simulink model "Quadruped_view"  (R2026a)
settings: Solver=ode23tb  StopTime=50
values from neighbouring files (symbols this model uses):
  a_amp = 0.03    [initializeRobotParameters.m]
  b_amp = 0.03    [initializeRobotParameters.m]
  dTheta = 20*pi/180    (= 0.349065850399)    [initializeRobotParameters.m]
  friction_force_max = mu_static * normal_force_max    [initializeRobotParameters.m]
  g = -9.81    [initializeRobotParameters.m]
  h_final = 0.2    [initializeRobotParameters.m]
  hip_eq_angle = 0    [initializeRobotParameters.m]
  init_ang_FL = d2r * quadrupedInverseKinematics(init_foot_disp_x,-init_body_height,l1,l2)    [initializeRobotParameters.m]
  init_ang_FR = init_ang_FL    [initializeRobotParameters.m]
  init_ang_RL = init_ang_FL    [initializeRobotParameters.m]
  init_ang_RR = init_ang_FL    [initializeRobotParameters.m]
  knee_eq_angle = 0    [initializeRobotParameters.m]
  l1 = 0.1422    [initializeRobotParameters.m]
  l2 = 0.115    [initializeRobotParameters.m]
  L_back = 0.305    [initializeRobotParameters.m]
  M = 1.318    [initializeRobotParameters.m]
  m1 = 0.17824    [initializeRobotParameters.m]
  m2 = 0.03558    [initializeRobotParameters.m]
  normal_force_max = ((M+4*m1+4*m2)*abs(g))/4    [initializeRobotParameters.m]
  period = 0.8    [initializeRobotParameters.m]
  pitch_max = 10 * d2r    (= 0.174532925199)    [initializeRobotParameters.m]
  q_hip_max = -30 * d2r    (= -0.523598775598)    [initializeRobotParameters.m]
  q_hip_min = -120 * d2r    (= -2.09439510239)    [initializeRobotParameters.m]
  q_knee_max = 140 * d2r    (= 2.44346095279)    [initializeRobotParameters.m]
  q_knee_min = 60 * d2r    (= 1.0471975512)    [initializeRobotParameters.m]
  roll_max = 10 * d2r    (= 0.174532925199)    [initializeRobotParameters.m]
  Tf = 10    [initializeRobotParameters.m]
  torso_dim = [L_back 0.04875 0.152]    [initializeRobotParameters.m]
  Tp = 0.15    [initializeRobotParameters.m]
  Ts = 0.025    [initializeRobotParameters.m]
  vx_max = 2.5    [initializeRobotParameters.m]
  vy_max = 2.5    [initializeRobotParameters.m]
  vz_max = 2.5    [initializeRobotParameters.m]
  w_max = 2*pi*60/60    (= 6.28318530718)    [initializeRobotParameters.m]
  y_init = init_body_height + foot_height    [initializeRobotParameters.m]
  y_max = l1*cos(q_hip_max) + l2*cos(q_hip_max+q_knee_min)    [initializeRobotParameters.m]
  y_min = 0.5    [initializeRobotParameters.m]
  yaw_max = 20 * d2r    (= 0.349065850399)    [initializeRobotParameters.m]
  z_max = 0.5    [initializeRobotParameters.m]
undefined symbols (not defined in the file or in its folder): Extr_Data_LinkEndHole, Extr_Data_Mesh, ground, joint, X, Y, Z
libraries: sm_lib x118, nesl_utility x54, simulink x4
(part 5 of 5)

== system Quadruped_view/Quadruped Robot/Leg RR/Lower Leg ==
  note: Geometry Only
  Cap F : sm_lib/Body Elements/Extruded Solid  ExtrusionType=General  PolygonNumSides=3  PolygonOuterRadius=1  PolygonOuterRadiusUnits=m  ExportEntireGeometry=off  ExtrusionCrossSection=Extr_Data_LinkEndHole(l2*0.1,l1*0.025,0.05*l2)  ExtrusionCrossSectionUnits=m  ExportConvexHullGeometry=off  ExtrusionLength=l2*0.1/3  ExtrusionLengthUnits=m  InertiaType=CalculateFromGeometry  BasedOnType=Density  Density=0  DensityUnits=kg/m^3  Mass=1  MassUnits=kg  CenterOfMass=[0 0 0]  CenterOfMassUnits=m  MomentsOfInertia=[1 1 1]  MomentsOfInertiaUnits=kg*m^2  ProductsOfInertia=[1 1 1]  ProductsOfInertiaUnits=kg*m^2  GraphicType=FromGeometry  MarkerShape=Sphere  MarkerSize=10  GraphicVisPropType=SimpleVisualProperties  GraphicDiffuseColor=[164 184 200]/255  GraphicOpacity=1.0  GraphicSpecularColor=[0.5 0.5 0.5 1.0]  GraphicAmbientColor=[0.15 0.15 0.15 1.0]  GraphicEmissiveColor=[0.0 0.0 0.0 1.0]  GraphicShininess=75  DoExposeReferenceFrame=on  SerializedFrames=<Frames/>
  Lower Leg : sm_lib/Body Elements/Brick Solid  BrickDimensions=[0.1 0.8 0.1]*l2  BrickDimensionsUnits=m  ExportEntireGeometry=off  InertiaType=Custom  BasedOnType=Density  Density=1000  DensityUnits=kg/m^3  Mass=m2  MassUnits=kg  CenterOfMass=link2_COM  CenterOfMassUnits=m  MomentsOfInertia=[1 1 1]*(1/12)*m2*l2*l2^2  MomentsOfInertiaUnits=kg*m^2  ProductsOfInertia=[1 1 1]*0  ProductsOfInertiaUnits=kg*m^2  GraphicType=FromGeometry  MarkerShape=Sphere  MarkerSize=10  GraphicVisPropType=SimpleVisualProperties  GraphicDiffuseColor=[164 184 200]/255  GraphicOpacity=1.0  GraphicSpecularColor=[0.5 0.5 0.5 1.0]  GraphicAmbientColor=[0.15 0.15 0.15 1.0]  GraphicEmissiveColor=[0.0 0.0 0.0 1.0]  GraphicShininess=75  DoExposeReferenceFrame=on  SerializedFrames=<Frames><Frame><Id>Frame1</Id><Value><Name>B</Name><Origin><Source>GeometricFeature</Source><FeatureName>-y surface</FeatureName></Origin><PrimaryAxis><DefinedDirection>+Z</DefinedDirection><Source>ReferenceFrame</Source><SourceDirection>+Z</SourceDirection><FeatureName></FeatureName></PrimaryAxis><SecondaryAxis><DefinedDirection>+X</DefinedDirection><Source>ReferenceFrame</Source><SourceDirection>+X</SourceDirection><FeatureName></FeatureName></SecondaryAxis></Value></Frame><Frame><Id>Frame2</Id><Value><Name>F</Name><Origin><Source>GeometricFeature</Source><FeatureName>+y surface</FeatureName></Origin><PrimaryAxis><DefinedDirection>+Z</DefinedDirection><Source>ReferenceFrame</Source><SourceDirection>+Z</SourceDirection><FeatureName></FeatureName></PrimaryAxis><SecondaryAxis><DefinedDirection>+X</DefinedDirection><Source>ReferenceFrame</Source><SourceDirection>+X</SourceDirection><FeatureName></FeatureName></SecondaryAxis></Value></Frame></Frames>
  Peg : sm_lib/Body Elements/Cylindrical Solid  CylinderRadius=0.05*l1  CylinderRadiusUnits=m  CylinderLength=0.05*l2  CylinderLengthUnits=m  ExportEntireGeometry=off  InertiaType=CalculateFromGeometry  BasedOnType=Density  Density=0  DensityUnits=kg/m^3  Mass=1  MassUnits=kg  CenterOfMass=[0 0 0]  CenterOfMassUnits=m  MomentsOfInertia=[1 1 1]  MomentsOfInertiaUnits=kg*m^2  ProductsOfInertia=[1 1 1]  ProductsOfInertiaUnits=kg*m^2  GraphicType=FromGeometry  MarkerShape=Sphere  MarkerSize=10  GraphicVisPropType=SimpleVisualProperties  GraphicDiffuseColor=[0.5 0.5 0.5]  GraphicOpacity=1.0  GraphicSpecularColor=[0.5 0.5 0.5 1.0]  GraphicAmbientColor=[0.15 0.15 0.15 1.0]  GraphicEmissiveColor=[0.0 0.0 0.0 1.0]  GraphicShininess=75  DoExposeReferenceFrame=off  SerializedFrames=<Frames><Frame><Id>Frame1</Id><Value><Name>B</Name><Origin><Source>GeometricFeature</Source><FeatureName>bottom surface</FeatureName></Origin><PrimaryAxis><DefinedDirection>+Z</DefinedDirection><Source>ReferenceFrame</Source><SourceDirection>+Z</SourceDirection><FeatureName></FeatureName></PrimaryAxis><SecondaryAxis><DefinedDirection>+X</DefinedDirection><Source>ReferenceFrame</Source><SourceDirection>+X</SourceDirection><FeatureName></FeatureName></SecondaryAxis></Value></Frame><Frame><Id>Frame2</Id><Value><Name>F</Name><Origin><Source>GeometricFeature</Source><FeatureName>top surface</FeatureName></Origin><PrimaryAxis><DefinedDirection>+Z</DefinedDirection><Source>ReferenceFrame</Source><SourceDirection>+Z</SourceDirection><FeatureName></FeatureName></PrimaryAxis><SecondaryAxis><DefinedDirection>+X</DefinedDirection><Source>ReferenceFrame</Source><SourceDirection>+X</SourceDirection><FeatureName></FeatureName></SecondaryAxis></Value></Frame></Frames>
  Pin : sm_lib/Body Elements/Cylindrical Solid  CylinderRadius=0.025*l1  CylinderRadiusUnits=m  CylinderLength=0.1*l2  CylinderLengthUnits=m  ExportEntireGeometry=off  InertiaType=CalculateFromGeometry  BasedOnType=Density  Density=0  DensityUnits=kg/m^3  Mass=1  MassUnits=kg  CenterOfMass=[0 0 0]  CenterOfMassUnits=m  MomentsOfInertia=[1 1 1]  MomentsOfInertiaUnits=kg*m^2  ProductsOfInertia=[1 1 1]  ProductsOfInertiaUnits=kg*m^2  GraphicType=FromGeometry  MarkerShape=Sphere  MarkerSize=10  GraphicVisPropType=SimpleVisualProperties  GraphicDiffuseColor=[164 184 200]/255  GraphicOpacity=1.0  GraphicSpecularColor=[0.5 0.5 0.5 1.0]  GraphicAmbientColor=[0.15 0.15 0.15 1.0]  GraphicEmissiveColor=[0.0 0.0 0.0 1.0]  GraphicShininess=75  DoExposeReferenceFrame=on  SerializedFrames=<Frames/>
  Sphere : sm_lib/Body Elements/Revolved Solid  RevolutionCrossSection=[sind(90:-1:0)' cosd(90:-1:0)']*l2*0.1/2  RevolutionCrossSectionUnits=m  RevolutionExtent=Full  RevolutionAngle=180  RevolutionAngleUnits=deg  ExportConvexHullGeometry=on  InertiaType=CalculateFromGeometry  BasedOnType=Density  Density=0  DensityUnits=kg/m^3  Mass=1  MassUnits=kg  CenterOfMass=[0 0 0]  CenterOfMassUnits=m  MomentsOfInertia=[1 1 1]  MomentsOfInertiaUnits=kg*m^2  ProductsOfInertia=[1 1 1]  ProductsOfInertiaUnits=kg*m^2  GraphicType=FromGeometry  MarkerShape=Sphere  MarkerSize=10  GraphicVisPropType=SimpleVisualProperties  GraphicDiffuseColor=[0.5 0.5 0.5]  GraphicOpacity=1.0  GraphicSpecularColor=[0.5 0.5 0.5 1.0]  GraphicAmbientColor=[0.15 0.15 0.15 1.0]  GraphicEmissiveColor=[0.0 0.0 0.0 1.0]  GraphicShininess=75  DoExposeReferenceFrame=on  SerializedFrames=<Frames/>
  Transform Cap F : sm_lib/Frames and Transforms/Rigid Transform  RotationMethod=StandardAxis  FollAlignAxisA=+X  BaseAlignAxisA=+Y  FollAlignAxisB=+Y  BaseAlignAxisB=+Z  RotationStandardAxis=+Z  RotationAngle=90  RotationAngleUnits=deg  RotationArbitraryAxis=[0 0 1]  RotationSequenceAxes=FollowerAxes  RotationSequence=XYX  RotationSequenceAngles=[0 0 0]  RotationSequenceAnglesUnits=deg  RotationMatrix=[1 0 0; 0 1 0; 0 0 1]  Quaternion=[1 0 0 0]  TranslationMethod=None  TranslationCartesianOffset=[0 0 0]  TranslationCartesianOffsetUnits=m  TranslationStandardAxis=+Z  TranslationStandardOffset=0  TranslationStandardOffsetUnits=m  TranslationROffset=0  TranslationROffsetUnits=m  TranslationThetaOffset=0  TranslationThetaOffsetUnits=deg  TranslationZOffset=0  TranslationZOffsetUnits=m
  Transform Peg : sm_lib/Frames and Transforms/Rigid Transform  RotationMethod=StandardAxis  FollAlignAxisA=+X  BaseAlignAxisA=+Y  FollAlignAxisB=+Y  BaseAlignAxisB=+Z  RotationStandardAxis=+X  RotationAngle=90  RotationAngleUnits=deg  RotationArbitraryAxis=[0 0 1]  RotationSequenceAxes=FollowerAxes  RotationSequence=XYX  RotationSequenceAngles=[0 0 0]  RotationSequenceAnglesUnits=deg  RotationMatrix=[1 0 0; 0 1 0; 0 0 1]  Quaternion=[1 0 0 0]  TranslationMethod=None  TranslationCartesianOffset=[0 0 0]  TranslationCartesianOffsetUnits=m  TranslationStandardAxis=+Z  TranslationStandardOffset=0  TranslationStandardOffsetUnits=m  TranslationROffset=0  TranslationROffsetUnits=m  TranslationThetaOffset=0  TranslationThetaOffsetUnits=deg  TranslationZOffset=0  TranslationZOffsetUnits=m
  Transform F : sm_lib/Frames and Transforms/Rigid Transform  RotationMethod=None  FollAlignAxisA=+X  BaseAlignAxisA=+Y  FollAlignAxisB=+Y  BaseAlignAxisB=+Z  RotationStandardAxis=+Z  RotationAngle=0.0  RotationAngleUnits=deg  RotationArbitraryAxis=[0 0 1]  RotationSequenceAxes=FollowerAxes  RotationSequence=XYX  RotationSequenceAngles=[0 0 0]  RotationSequenceAnglesUnits=deg  RotationMatrix=[1 0 0; 0 1 0; 0 0 1]  Quaternion=[1 0 0 0]  TranslationMethod=StandardAxis  TranslationCartesianOffset=[0 0 0]  TranslationCartesianOffsetUnits=m  TranslationStandardAxis=+Y  TranslationStandardOffset=l2/2  TranslationStandardOffsetUnits=m  TranslationROffset=0  TranslationROffsetUnits=m  TranslationThetaOffset=0  TranslationThetaOffsetUnits=deg  TranslationZOffset=0  TranslationZOffsetUnits=m
  Transform R : sm_lib/Frames and Transforms/Rigid Transform  RotationMethod=None  FollAlignAxisA=+X  BaseAlignAxisA=+Y  FollAlignAxisB=+Y  BaseAlignAxisB=+Z  RotationStandardAxis=+Z  RotationAngle=0.0  RotationAngleUnits=deg  RotationArbitraryAxis=[0 0 1]  RotationSequenceAxes=FollowerAxes  RotationSequence=XYX  RotationSequenceAngles=[0 0 0]  RotationSequenceAnglesUnits=deg  RotationMatrix=[1 0 0; 0 1 0; 0 0 1]  Quaternion=[1 0 0 0]  TranslationMethod=StandardAxis  TranslationCartesianOffset=[0 0 0]  TranslationCartesianOffsetUnits=m  TranslationStandardAxis=+Y  TranslationStandardOffset=l1/2  TranslationStandardOffsetUnits=m  TranslationROffset=0  TranslationROffsetUnits=m  TranslationThetaOffset=0  TranslationThetaOffsetUnits=deg  TranslationZOffset=0  TranslationZOffsetUnits=m
  F : PMIOPort  Side=Right
  SG : PMIOPort  Port=2  Side=Left
  B : PMIOPort  Port=3  Side=Left
  connections:
  Peg/RConn1 -- Sphere/RConn1
  Peg/LConn1 -- Transform Peg/RConn1
  Transform Peg/LConn1 -- Lower Leg/LConn1
  Cap F/RConn1 -- Transform Cap F/RConn1
  Transform Cap F/LConn1 -- Lower Leg/LConn2
  Transform F/LConn1 -- Transform R/RConn1 -- Lower Leg/RConn1
  Transform F/RConn1 -- Pin/RConn1 -- F/RConn1
  B/RConn1 -- Transform R/LConn1
  SG/RConn1 -- Sphere/LConn1

== system Quadruped_view/Quadruped Robot/Leg RR/Rotary Displacement and Speed Sensor - Hip ==
  Bus Creator : BusCreator  Inputs=2
  Gain : Gain  Gain=-1
  Gain1 : Gain  Gain=-1
  PS-Simulink Converter : nesl_utility/PS-Simulink Converter  PhysicalDomain=network_engine_domain  SubClassName=ps_output  LeftPortType=input  RightPortType=output  PseudoPeriodic=off  Frequencies=[]  VectorFormat=1-D array  Unit=1  AffineConversion=off
  PS-Simulink Converter1 : nesl_utility/PS-Simulink Converter  PhysicalDomain=network_engine_domain  SubClassName=ps_output  LeftPortType=input  RightPortType=output  PseudoPeriodic=off  Frequencies=[]  VectorFormat=1-D array  Unit=1  AffineConversion=off
  q : PMIOPort  Side=Left
  w : PMIOPort  Port=2  Side=Left
  data : Outport  VectorParamsAs1DForOutWhenUnconnected=off
  wires:
  Gain1/1 -> Bus Creator/2  "vel"
  Gain/1 -> Bus Creator/1  "ang"
  PS-Simulink Converter1/1 -> Gain1/1
  PS-Simulink Converter/1 -> Gain/1
  Bus Creator/1 -> data/1
  connections:
  PS-Simulink Converter1/LConn1 -- w/RConn1
  PS-Simulink Converter/LConn1 -- q/RConn1

== system Quadruped_view/Quadruped Robot/Leg RR/Rotary Displacement and Speed Sensor - Knee ==
  Bus Creator : BusCreator  Inputs=2
  Gain : Gain  Gain=-1  OutDataTypeStr=Inherit: Same as input
  Gain1 : Gain  Gain=-1  OutDataTypeStr=Inherit: Same as input
  PS-Simulink Converter : nesl_utility/PS-Simulink Converter  PhysicalDomain=network_engine_domain  SubClassName=ps_output  LeftPortType=input  RightPortType=output  PseudoPeriodic=off  Frequencies=[]  VectorFormat=1-D array  Unit=1  AffineConversion=off
  PS-Simulink Converter1 : nesl_utility/PS-Simulink Converter  PhysicalDomain=network_engine_domain  SubClassName=ps_output  LeftPortType=input  RightPortType=output  PseudoPeriodic=off  Frequencies=[]  VectorFormat=1-D array  Unit=1  AffineConversion=off
  q : PMIOPort  Side=Left
  w : PMIOPort  Port=2  Side=Left
  data : Outport  VectorParamsAs1DForOutWhenUnconnected=off
  wires:
  Gain1/1 -> Bus Creator/2  "vel"
  Gain/1 -> Bus Creator/1  "ang"
  Bus Creator/1 -> data/1
  PS-Simulink Converter/1 -> Gain/1
  PS-Simulink Converter1/1 -> Gain1/1
  connections:
  PS-Simulink Converter/LConn1 -- q/RConn1
  PS-Simulink Converter1/LConn1 -- w/RConn1

== system Quadruped_view/Quadruped Robot/Leg RR/Upper Leg ==
  note: Geometry Only
  Cap B Left : sm_lib/Body Elements/Extruded Solid  ExtrusionType=General  PolygonNumSides=3  PolygonOuterRadius=1  PolygonOuterRadiusUnits=m  ExportEntireGeometry=off  ExtrusionCrossSection=Extr_Data_LinkEndHole(l1*0.1,l1*0.025,0.05*l1)  ExtrusionCrossSectionUnits=m  ExportConvexHullGeometry=off  ExtrusionLength=l1*0.1/3  ExtrusionLengthUnits=m  InertiaType=CalculateFromGeometry  BasedOnType=Density  Density=0  DensityUnits=kg/m^3  Mass=1  MassUnits=kg  CenterOfMass=[0 0 0]  CenterOfMassUnits=m  MomentsOfInertia=[1 1 1]  MomentsOfInertiaUnits=kg*m^2  ProductsOfInertia=[1 1 1]  ProductsOfInertiaUnits=kg*m^2  GraphicType=FromGeometry  MarkerShape=Sphere  MarkerSize=10  GraphicVisPropType=SimpleVisualProperties  GraphicDiffuseColor=[0.2 0.4 0.6]  GraphicOpacity=1.0  GraphicSpecularColor=[0.5 0.5 0.5 1.0]  GraphicAmbientColor=[0.15 0.15 0.15 1.0]  GraphicEmissiveColor=[0.0 0.0 0.0 1.0]  GraphicShininess=75  DoExposeReferenceFrame=on  SerializedFrames=<Frames/>
  Cap B Right : sm_lib/Body Elements/Extruded Solid  ExtrusionType=General  PolygonNumSides=3  PolygonOuterRadius=1  PolygonOuterRadiusUnits=m  ExportEntireGeometry=off  ExtrusionCrossSection=Extr_Data_LinkEndHole(l1*0.1,l1*0.025,0.05*l1)  ExtrusionCrossSectionUnits=m  ExportConvexHullGeometry=off  ExtrusionLength=l1*0.1/3  ExtrusionLengthUnits=m  InertiaType=CalculateFromGeometry  BasedOnType=Density  Density=0  DensityUnits=kg/m^3  Mass=1  MassUnits=kg  CenterOfMass=[0 0 0]  CenterOfMassUnits=m  MomentsOfInertia=[1 1 1]  MomentsOfInertiaUnits=kg*m^2  ProductsOfInertia=[1 1 1]  ProductsOfInertiaUnits=kg*m^2  GraphicType=FromGeometry  MarkerShape=Sphere  MarkerSize=10  GraphicVisPropType=SimpleVisualProperties  GraphicDiffuseColor=[0.2 0.4 0.6]  GraphicOpacity=1.0  GraphicSpecularColor=[0.5 0.5 0.5 1.0]  GraphicAmbientColor=[0.15 0.15 0.15 1.0]  GraphicEmissiveColor=[0.0 0.0 0.0 1.0]  GraphicShininess=75  DoExposeReferenceFrame=on  SerializedFrames=<Frames/>
  Cap F : sm_lib/Body Elements/Extruded Solid  ExtrusionType=General  PolygonNumSides=3  PolygonOuterRadius=1  PolygonOuterRadiusUnits=m  ExportEntireGeometry=off  ExtrusionCrossSection=Extr_Data_LinkEndHole(l1*0.1,l1*0.025,0.05*l1)  ExtrusionCrossSectionUnits=m  ExportConvexHullGeometry=off  ExtrusionLength=l1*0.1  ExtrusionLengthUnits=m  InertiaType=CalculateFromGeometry  BasedOnType=Density  Density=0  DensityUnits=kg/m^3  Mass=1  MassUnits=kg  CenterOfMass=[0 0 0]  CenterOfMassUnits=m  MomentsOfInertia=[1 1 1]  MomentsOfInertiaUnits=kg*m^2  ProductsOfInertia=[1 1 1]  ProductsOfInertiaUnits=kg*m^2  GraphicType=FromGeometry  MarkerShape=Sphere  MarkerSize=10  GraphicVisPropType=SimpleVisualProperties  GraphicDiffuseColor=[0.2 0.4 0.6]  GraphicOpacity=1.0  GraphicSpecularColor=[0.5 0.5 0.5 1.0]  GraphicAmbientColor=[0.15 0.15 0.15 1.0]  GraphicEmissiveColor=[0.0 0.0 0.0 1.0]  GraphicShininess=75  DoExposeReferenceFrame=on  SerializedFrames=<Frames/>
  Rigid Transform : sm_lib/Frames and Transforms/Rigid Transform  RotationMethod=StandardAxis  FollAlignAxisA=+X  BaseAlignAxisA=+Y  FollAlignAxisB=+Y  BaseAlignAxisB=+Z  RotationStandardAxis=+Z  RotationAngle=-90  RotationAngleUnits=deg  RotationArbitraryAxis=[0 0 1]  RotationSequenceAxes=FollowerAxes  RotationSequence=XYX  RotationSequenceAngles=[0 0 0]  RotationSequenceAnglesUnits=deg  RotationMatrix=[1 0 0; 0 1 0; 0 0 1]  Quaternion=[1 0 0 0]  TranslationMethod=StandardAxis  TranslationCartesianOffset=[0 0 0]  TranslationCartesianOffsetUnits=m  TranslationStandardAxis=+Z  TranslationStandardOffset=0.1*l1/3  TranslationStandardOffsetUnits=m  TranslationROffset=0  TranslationROffsetUnits=m  TranslationThetaOffset=0  TranslationThetaOffsetUnits=deg  TranslationZOffset=0  TranslationZOffsetUnits=m
  Transform Cap F : sm_lib/Frames and Transforms/Rigid Transform  RotationMethod=StandardAxis  FollAlignAxisA=+X  BaseAlignAxisA=+Y  FollAlignAxisB=+Y  BaseAlignAxisB=+Z  RotationStandardAxis=+Z  RotationAngle=90  RotationAngleUnits=deg  RotationArbitraryAxis=[0 0 1]  RotationSequenceAxes=FollowerAxes  RotationSequence=XYX  RotationSequenceAngles=[0 0 0]  RotationSequenceAnglesUnits=deg  RotationMatrix=[1 0 0; 0 1 0; 0 0 1]  Quaternion=[1 0 0 0]  TranslationMethod=None  TranslationCartesianOffset=[0 0 0]  TranslationCartesianOffsetUnits=m  TranslationStandardAxis=+Z  TranslationStandardOffset=0  TranslationStandardOffsetUnits=m  TranslationROffset=0  TranslationROffsetUnits=m  TranslationThetaOffset=0  TranslationThetaOffsetUnits=deg  TranslationZOffset=0  TranslationZOffsetUnits=m
  Transform F : sm_lib/Frames and Transforms/Rigid Transform  RotationMethod=None  FollAlignAxisA=+X  BaseAlignAxisA=+Y  FollAlignAxisB=+Y  BaseAlignAxisB=+Z  RotationStandardAxis=+Z  RotationAngle=0.0  RotationAngleUnits=deg  RotationArbitraryAxis=[0 0 1]  RotationSequenceAxes=FollowerAxes  RotationSequence=XYX  RotationSequenceAngles=[0 0 0]  RotationSequenceAnglesUnits=deg  RotationMatrix=[1 0 0; 0 1 0; 0 0 1]  Quaternion=[1 0 0 0]  TranslationMethod=StandardAxis  TranslationCartesianOffset=[0 0 0]  TranslationCartesianOffsetUnits=m  TranslationStandardAxis=+Y  TranslationStandardOffset=l1/2  TranslationStandardOffsetUnits=m  TranslationROffset=0  TranslationROffsetUnits=m  TranslationThetaOffset=0  TranslationThetaOffsetUnits=deg  TranslationZOffset=0  TranslationZOffsetUnits=m
  Transform R : sm_lib/Frames and Transforms/Rigid Transform  RotationMethod=None  FollAlignAxisA=+X  BaseAlignAxisA=+Y  FollAlignAxisB=+Y  BaseAlignAxisB=+Z  RotationStandardAxis=+Z  RotationAngle=0.0  RotationAngleUnits=deg  RotationArbitraryAxis=[0 0 1]  RotationSequenceAxes=FollowerAxes  RotationSequence=XYX  RotationSequenceAngles=[0 0 0]  RotationSequenceAnglesUnits=deg  RotationMatrix=[1 0 0; 0 1 0; 0 0 1]  Quaternion=[1 0 0 0]  TranslationMethod=StandardAxis  TranslationCartesianOffset=[0 0 0]  TranslationCartesianOffsetUnits=m  TranslationStandardAxis=+Y  TranslationStandardOffset=l1/2  TranslationStandardOffsetUnits=m  TranslationROffset=0  TranslationROffsetUnits=m  TranslationThetaOffset=0  TranslationThetaOffsetUnits=deg  TranslationZOffset=0  TranslationZOffsetUnits=m
  "Transform Stem " : sm_lib/Frames and Transforms/Rigid Transform  RotationMethod=StandardAxis  FollAlignAxisA=+X  BaseAlignAxisA=+Y  FollAlignAxisB=+Y  BaseAlignAxisB=+Z  RotationStandardAxis=+Z  RotationAngle=-90  RotationAngleUnits=deg  RotationArbitraryAxis=[0 0 1]  RotationSequenceAxes=FollowerAxes  RotationSequence=XYX  RotationSequenceAngles=[0 0 0]  RotationSequenceAnglesUnits=deg  RotationMatrix=[1 0 0; 0 1 0; 0 0 1]  Quaternion=[1 0 0 0]  TranslationMethod=StandardAxis  TranslationCartesianOffset=[0 0 0]  TranslationCartesianOffsetUnits=m  TranslationStandardAxis=+Z  TranslationStandardOffset=-0.1*l1/3  TranslationStandardOffsetUnits=m  TranslationROffset=0  TranslationROffsetUnits=m  TranslationThetaOffset=0  TranslationThetaOffsetUnits=deg  TranslationZOffset=0  TranslationZOffsetUnits=m
  Upper Leg : sm_lib/Body Elements/Brick Solid  BrickDimensions=[0.1 0.8 0.1]*l1  BrickDimensionsUnits=m  ExportEntireGeometry=off  InertiaType=Custom  BasedOnType=Density  Density=1000  DensityUnits=kg/m^3  Mass=m1  MassUnits=kg  CenterOfMass=link1_COM  CenterOfMassUnits=m  MomentsOfInertia=[1 1 1]*(1/12)*m1*l1*l1^2  MomentsOfInertiaUnits=kg*m^2  ProductsOfInertia=[1 1 1]*0  ProductsOfInertiaUnits=kg*m^2  GraphicType=FromGeometry  MarkerShape=Sphere  MarkerSize=10  GraphicVisPropType=SimpleVisualProperties  GraphicDiffuseColor=[0.2 0.4 0.6]  GraphicOpacity=1.0  GraphicSpecularColor=[0.5 0.5 0.5 1.0]  GraphicAmbientColor=[0.15 0.15 0.15 1.0]  GraphicEmissiveColor=[0.0 0.0 0.0 1.0]  GraphicShininess=75  DoExposeReferenceFrame=on  SerializedFrames=<Frames><Frame><Id>Frame1</Id><Value><Name>B</Name><Origin><Source>GeometricFeature</Source><FeatureName>-y surface</FeatureName></Origin><PrimaryAxis><DefinedDirection>+Z</DefinedDirection><Source>ReferenceFrame</Source><SourceDirection>+Z</SourceDirection><FeatureName></FeatureName></PrimaryAxis><SecondaryAxis><DefinedDirection>+X</DefinedDirection><Source>ReferenceFrame</Source><SourceDirection>+X</SourceDirection><FeatureName></FeatureName></SecondaryAxis></Value></Frame><Frame><Id>Frame2</Id><Value><Name>F</Name><Origin><Source>GeometricFeature</Source><FeatureName>+y surface</FeatureName></Origin><PrimaryAxis><DefinedDirection>+Z</DefinedDirection><Source>ReferenceFrame</Source><SourceDirection>+Z</SourceDirection><FeatureName></FeatureName></PrimaryAxis><SecondaryAxis><DefinedDirection>+X</DefinedDirection><Source>ReferenceFrame</Source><SourceDirection>+X</SourceDirection><FeatureName></FeatureName></SecondaryAxis></Value></Frame></Frames>
  F : PMIOPort  Side=Right
  B : PMIOPort  Port=2  Side=Left
  connections:
  Transform Cap F/LConn1 -- Upper Leg/LConn2
  "Transform Stem "/RConn1 -- Cap B Left/RConn1
  Upper Leg/LConn1 -- "Transform Stem "/LConn1 -- Rigid Transform/LConn1
  Cap F/RConn1 -- Transform Cap F/RConn1
  Cap B Right/RConn1 -- Rigid Transform/RConn1
  Transform F/LConn1 -- Transform R/RConn1 -- Upper Leg/RConn1
  Transform F/RConn1 -- F/RConn1
  B/RConn1 -- Transform R/LConn1

== system Quadruped_view/Quadruped Robot/Sensors/Leg Sensors ==
  FL : Inport
  FR : Inport  Port=2
  RL : Inport  Port=3
  RR : Inport  Port=4
  Rate Transition{,1..3} (4 alike) : RateTransition  Commented=through  OutPortSampleTime=Ts
  FLbus : Outport  VectorParamsAs1DForOutWhenUnconnected=off
  FRbus : Outport  Port=2  VectorParamsAs1DForOutWhenUnconnected=off
  RLbus : Outport  Port=3  VectorParamsAs1DForOutWhenUnconnected=off
  RRbus : Outport  Port=4  VectorParamsAs1DForOutWhenUnconnected=off
  wires:
  FL/1 -> Rate Transition/1
  FR/1 -> Rate Transition1/1
  Rate Transition2/1 -> RLbus/1
  RL/1 -> Rate Transition2/1
  Rate Transition3/1 -> RRbus/1
  RR/1 -> Rate Transition3/1
  Rate Transition/1 -> FLbus/1
  Rate Transition1/1 -> FRbus/1

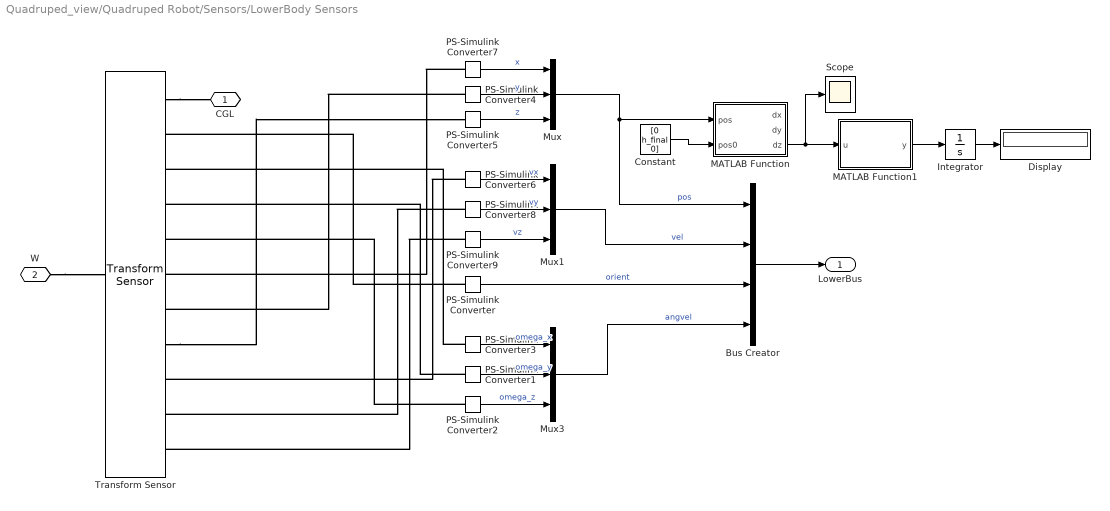
== system Quadruped_view/Quadruped Robot/Sensors/LowerBody Sensors ==
  Bus Creator : BusCreator  Inputs=4
  Constant : Constant  Value=[0 h_final 0]
  Display : Display
  Integrator : Integrator
  MATLAB Function : MATLAB Function  TreatAsAtomicUnit=on
  MATLAB Function1 : MATLAB Function  TreatAsAtomicUnit=on
  Mux : Mux  Inputs=3
  Mux1 : Mux  Inputs=3
  Mux3 : Mux  Inputs=3
  PS-Simulink Converter{,1..9} (10 alike) : nesl_utility/PS-Simulink Converter  PhysicalDomain=network_engine_domain  SubClassName=ps_output  LeftPortType=input  RightPortType=output  PseudoPeriodic=off  Frequencies=[]  VectorFormat=1-D array  Unit=1  AffineConversion=off
  Scope : Scope
      settings: ActiveDisplayYMinimum=-0.059294290574294091  ActiveDisplayYMaximum=0.048854241539892873
  Transform Sensor : sm_lib/Frames and Transforms/Transform Sensor  MeasurementFrame=World  RotationSequence=XYX  SenseAngle=off  SenseAxis=off  SenseQ=on  SenseR=off  SenseRotationSequence=off  SenseOmegaX=on  SenseOmegaY=on  SenseOmegaZ=on  SenseOmega=off  SenseQDot=off  SenseRDot=off  SenseRotationSequenceDot=off  SenseAlphaX=off  SenseAlphaY=off  SenseAlphaZ=off  SenseAlpha=off  SenseQDDot=off  SenseRDDot=off  SenseX=on  SenseY=on  SenseZ=on  SenseXYZ=off  SenseRad=off  SenseAzim=off  SenseDist=off  SenseInc=off  SenseXDot=on  SenseYDot=on  SenseZDot=on  SenseXYZDot=off  SenseRadDot=off  SenseAzimDot=off  SenseDistDot=off  SenseIncDot=off  SenseXDDot=off  SenseYDDot=off  SenseZDDot=off  SenseXYZDDot=off  SenseRadDDot=off  SenseAzimDDot=off  SenseDistDDot=off  SenseIncDDot=off
  CGL : PMIOPort  Side=Left
  W : PMIOPort  Port=2  Side=Left
  LowerBus : Outport  VectorParamsAs1DForOutWhenUnconnected=off
  wires:
  Bus Creator/1 -> LowerBus/1
  PS-Simulink Converter3/1 -> Mux3/1  "omega_x"
  PS-Simulink Converter2/1 -> Mux3/3  "omega_z"
  PS-Simulink Converter1/1 -> Mux3/2  "omega_y"
  PS-Simulink Converter6/1 -> Mux1/1  "vx"
  PS-Simulink Converter4/1 -> Mux/2  "y"
  PS-Simulink Converter7/1 -> Mux/1  "x"
  PS-Simulink Converter5/1 -> Mux/3  "z"
  PS-Simulink Converter8/1 -> Mux1/2  "vy"
  PS-Simulink Converter9/1 -> Mux1/3  "vz"
  Mux/1 -> MATLAB Function/1(pos), Bus Creator/1  "pos"
  Mux1/1 -> Bus Creator/2  "vel"
  Mux3/1 -> Bus Creator/4  "angvel"
  PS-Simulink Converter/1 -> Bus Creator/3  "orient"
  Constant/1 -> MATLAB Function/2(pos0)
  MATLAB Function/3(dz) -> Scope/1, MATLAB Function1/1(u)
  MATLAB Function1/1(y) -> Integrator/1
  Integrator/1 -> Display/1
  connections:
  Transform Sensor/RConn1 -- CGL/RConn1
  W/RConn1 -- Transform Sensor/LConn1
  PS-Simulink Converter6/LConn1 -- Transform Sensor/RConn9
  PS-Simulink Converter3/LConn1 -- Transform Sensor/RConn3
  PS-Simulink Converter1/LConn1 -- Transform Sensor/RConn4
  PS-Simulink Converter2/LConn1 -- Transform Sensor/RConn5
  PS-Simulink Converter4/LConn1 -- Transform Sensor/RConn7
  Transform Sensor/RConn8 -- PS-Simulink Converter5/LConn1
  PS-Simulink Converter7/LConn1 -- Transform Sensor/RConn6
  PS-Simulink Converter/LConn1 -- Transform Sensor/RConn2
  PS-Simulink Converter8/LConn1 -- Transform Sensor/RConn10
  PS-Simulink Converter9/LConn1 -- Transform Sensor/RConn11

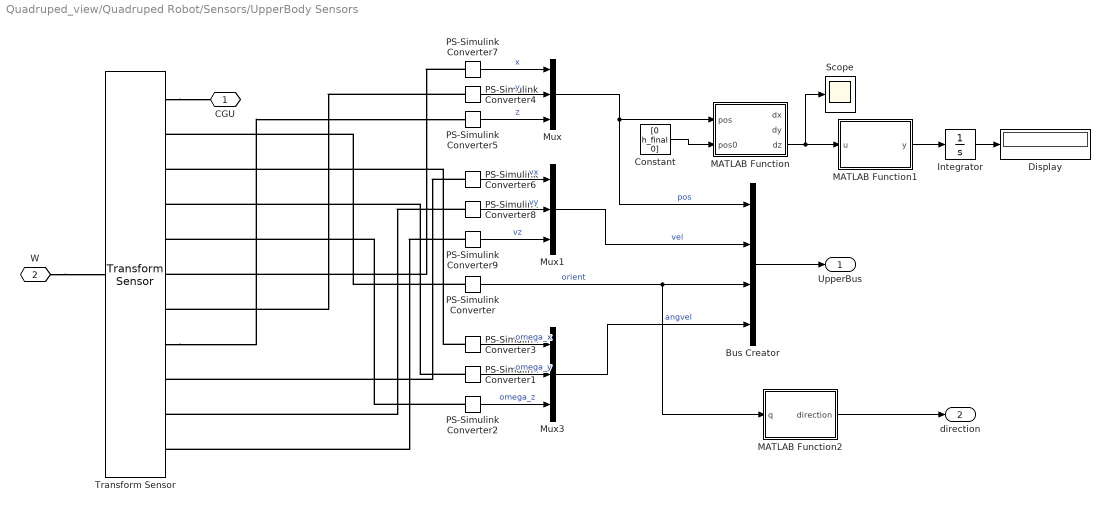
== system Quadruped_view/Quadruped Robot/Sensors/UpperBody Sensors ==
  Bus Creator : BusCreator  Inputs=4
  Constant : Constant  Value=[0 h_final 0]
  Display : Display
  Integrator : Integrator
  MATLAB Function : MATLAB Function  TreatAsAtomicUnit=on
  MATLAB Function1 : MATLAB Function  TreatAsAtomicUnit=on
  MATLAB Function2 : MATLAB Function  TreatAsAtomicUnit=on
  Mux : Mux  Inputs=3
  Mux1 : Mux  Inputs=3
  Mux3 : Mux  Inputs=3
  PS-Simulink Converter{,1..9} (10 alike) : nesl_utility/PS-Simulink Converter  PhysicalDomain=network_engine_domain  SubClassName=ps_output  LeftPortType=input  RightPortType=output  PseudoPeriodic=off  Frequencies=[]  VectorFormat=1-D array  Unit=1  AffineConversion=off
  Scope : Scope
      settings: ActiveDisplayYMinimum=-0.059294290574294091  ActiveDisplayYMaximum=0.048854241539892873
  Transform Sensor : sm_lib/Frames and Transforms/Transform Sensor  MeasurementFrame=World  RotationSequence=XYX  SenseAngle=off  SenseAxis=off  SenseQ=on  SenseR=off  SenseRotationSequence=off  SenseOmegaX=on  SenseOmegaY=on  SenseOmegaZ=on  SenseOmega=off  SenseQDot=off  SenseRDot=off  SenseRotationSequenceDot=off  SenseAlphaX=off  SenseAlphaY=off  SenseAlphaZ=off  SenseAlpha=off  SenseQDDot=off  SenseRDDot=off  SenseX=on  SenseY=on  SenseZ=on  SenseXYZ=off  SenseRad=off  SenseAzim=off  SenseDist=off  SenseInc=off  SenseXDot=on  SenseYDot=on  SenseZDot=on  SenseXYZDot=off  SenseRadDot=off  SenseAzimDot=off  SenseDistDot=off  SenseIncDot=off  SenseXDDot=off  SenseYDDot=off  SenseZDDot=off  SenseXYZDDot=off  SenseRadDDot=off  SenseAzimDDot=off  SenseDistDDot=off  SenseIncDDot=off
  CGU : PMIOPort  Side=Left
  W : PMIOPort  Port=2  Side=Left
  UpperBus : Outport  VectorParamsAs1DForOutWhenUnconnected=off
  direction : Outport  Port=2
  wires:
  Bus Creator/1 -> UpperBus/1
  PS-Simulink Converter3/1 -> Mux3/1  "omega_x"
  PS-Simulink Converter2/1 -> Mux3/3  "omega_z"
  PS-Simulink Converter1/1 -> Mux3/2  "omega_y"
  PS-Simulink Converter6/1 -> Mux1/1  "vx"
  PS-Simulink Converter4/1 -> Mux/2  "y"
  PS-Simulink Converter7/1 -> Mux/1  "x"
  PS-Simulink Converter5/1 -> Mux/3  "z"
  PS-Simulink Converter8/1 -> Mux1/2  "vy"
  PS-Simulink Converter9/1 -> Mux1/3  "vz"
  Mux/1 -> MATLAB Function/1(pos), Bus Creator/1  "pos"
  Mux1/1 -> Bus Creator/2  "vel"
  Mux3/1 -> Bus Creator/4  "angvel"
  PS-Simulink Converter/1 -> MATLAB Function2/1(q), Bus Creator/3  "orient"
  Constant/1 -> MATLAB Function/2(pos0)
  MATLAB Function/3(dz) -> Scope/1, MATLAB Function1/1(u)
  MATLAB Function1/1(y) -> Integrator/1
  Integrator/1 -> Display/1
  MATLAB Function2/1(direction) -> direction/1
  connections:
  Transform Sensor/RConn1 -- CGU/RConn1
  W/RConn1 -- Transform Sensor/LConn1
  PS-Simulink Converter6/LConn1 -- Transform Sensor/RConn9
  PS-Simulink Converter3/LConn1 -- Transform Sensor/RConn3
  PS-Simulink Converter1/LConn1 -- Transform Sensor/RConn4
  PS-Simulink Converter2/LConn1 -- Transform Sensor/RConn5
  PS-Simulink Converter4/LConn1 -- Transform Sensor/RConn7
  Transform Sensor/RConn8 -- PS-Simulink Converter5/LConn1
  PS-Simulink Converter7/LConn1 -- Transform Sensor/RConn6
  PS-Simulink Converter/LConn1 -- Transform Sensor/RConn2
  PS-Simulink Converter8/LConn1 -- Transform Sensor/RConn10
  PS-Simulink Converter9/LConn1 -- Transform Sensor/RConn11

== system Quadruped_view/Quadruped Robot/Sensors/Visualization Camera ==
  Camera : sm_lib/Body Elements/Graphic  GraphicType=Marker  MarkerShape=Frame  MarkerSize=10  GraphicVisPropType=SimpleVisualProperties  GraphicDiffuseColor=[0.5 0.5 0.5]  GraphicOpacity=1.0  GraphicSpecularColor=[0.5 0.5 0.5 1.0]  GraphicAmbientColor=[0.15 0.15 0.15 1.0]  GraphicEmissiveColor=[0.0 0.0 0.0 1.0]  GraphicShininess=75
  Rigid Transform : sm_lib/Frames and Transforms/Rigid Transform  RotationMethod=None  FollAlignAxisA=+X  BaseAlignAxisA=+Y  FollAlignAxisB=+Y  BaseAlignAxisB=+Z  RotationStandardAxis=+Z  RotationAngle=0.0  RotationAngleUnits=deg  RotationArbitraryAxis=[0 0 1]  RotationSequenceAxes=FollowerAxes  RotationSequence=XYX  RotationSequenceAngles=[0 0 0]  RotationSequenceAnglesUnits=deg  RotationMatrix=[1 0 0; 0 1 0; 0 0 1]  Quaternion=[1 0 0 0]  TranslationMethod=StandardAxis  TranslationCartesianOffset=[0 0 0]  TranslationCartesianOffsetUnits=m  TranslationStandardAxis=+Z  TranslationStandardOffset=3  TranslationStandardOffsetUnits=m  TranslationROffset=0  TranslationROffsetUnits=m  TranslationThetaOffset=0  TranslationThetaOffsetUnits=deg  TranslationZOffset=0  TranslationZOffsetUnits=m
  B : PMIOPort  Side=Left
  connections:
  Camera/RConn1 -- Rigid Transform/RConn1
  Rigid Transform/LConn1 -- B/RConn1

== matlab function Quadruped_view/Reward/MATLAB Function ==
  data: q input; e output
function e = quatToEuler(q)

% Normalize the quaternions
q = bsxfun(@times, q, 1./sqrt(sum(q.^2,1)));

qw = q(1);
qx = q(2);
qy = q(3);
qz = q(4);

% Pre-allocate output
%e = zeros(3, 1, 'like', q);

aSinInput = -2*(qx.*qz-qw.*qy);
aSinInput(aSinInput > 1) = 1;
aSinInput(aSinInput < -1) = -1;

e = [ atan2( 2*(qx.*qy+qw.*qz), qw.^2 + qx.^2 - qy.^2 - qz.^2 ); ...
    asin( aSinInput ); ...
    atan2( 2*(qy.*qz+qw.*qx), qw.^2 - qx.^2 - qy.^2 + qz.^2 )];

% roll = atan2(2*(q0*q1+q2*q3),(1-2*(q1^2+q2^2)));  %phi
% yaw = asin(2*(q0*q2-q3*q1));
% pitch = atan2(2*(q0*q3+q1*q2),(1-2*(q2^2+q3^2)));
% 
% e = [pitch; yaw; roll];  % ZYX

== matlab function Quadruped_view/Check If Done/MATLAB Function ==
  data: q input; R output
function R = quatToRotM(q)
% Quaternion to Rotation matrix conversion
% Source: https://en.wikipedia.org/wiki/Quaternions_and_spatial_rotation#Quaternion-derived_rotation_matrix

% Normalize the quaternions
q = bsxfun(@times, q, 1./sqrt(sum(q.^2,1)));

q0 = q(1);
q1 = q(2);
q2 = q(3);
q3 = q(4);

r11 = 1 - 2*(q2^2+q3^2);
r12 = 2*(q1*q2-q0*q3);
r13 = 2*(q0*q2+q1*q3);
r21 = 2*(q1*q2+q0*q3);
r22 = 1 - 2*(q1^2+q3^2);
r23 = 2*(q2*q3-q0*q1);
r31 = 2*(q1*q3-q0*q2);
r32 = 2*(q0*q1+q2*q3);
r33 = 1 - 2*(q1^2+q2^2);

R = [r11 r12 r13; r21 r22 r23; r31 r32 r33];

== matlab function Quadruped_view/MATLAB Function ==
  data: t input; angles output; T input; a_amp input; b_amp input
function angles = fcn(t,T,a_amp,b_amp)
h_final=0.2;
l1 = 0.1422;  % Link #1 length (m)
l2 = 0.115;  % Link #2 length (m)
w=2*pi/T;
a1=-a_amp*sin(w*t);
a2=a_amp*sin(w*t);
b1=-h_final-b_amp*sin(w*t)/2;
b2=-h_final+b_amp*sin(w*t)/2;

q1 = (pi/180)*quadrupedInverseKinematics(a1,b1,l1,l2);
q2 = (pi/180)*quadrupedInverseKinematics(a2,b2,l1,l2);
angles=[q1 q2 q2 q1];
end

== matlab function Quadruped_view/Quadruped Robot/Sensors/UpperBody Sensors/MATLAB Function ==
  data: pos input; dx output; pos0 input; dy output; dz output
function [dx,dy,dz] = fcn(pos,pos0)
dx = pos(1) - pos0(1);
dy = pos(2) - pos0(2);
dz = pos(3) - pos0(3);
end

== matlab function Quadruped_view/Quadruped Robot/Sensors/UpperBody Sensors/MATLAB Function1 ==
  data: u input; y output
function y = fcn(u)
y = u^2;
end

== matlab function Quadruped_view/Quadruped Robot/Sensors/LowerBody Sensors/MATLAB Function ==
  data: pos input; dx output; pos0 input; dy output; dz output
function [dx,dy,dz] = fcn(pos,pos0)
dx = pos(1) - pos0(1);
dy = pos(2) - pos0(2);
dz = pos(3) - pos0(3);
end

== matlab function Quadruped_view/Quadruped Robot/Sensors/LowerBody Sensors/MATLAB Function1 ==
  data: u input; y output
function y = fcn(u)
y = u^2;
end

== matlab function Quadruped_view/Quadruped Robot/MATLAB Function ==
  data: u input; y output; l input
function y = contact(u,l)
if u==0&&l==1
    y=1;
elseif u==1&&l==0
    y=-1;
else
    y=0;
end

== matlab function Quadruped_view/Quadruped Robot/Body/MATLAB Function ==
  data: direction input; c input; qcmd output; dTheta input; Tp input; Ts input
function qcmd = waistMove(direction,c,dTheta,Tp,Ts)
persistent cPrev elapsed qStart qTarget active

if isempty(cPrev)
    cPrev = 0;
    elapsed = 0;
    qStart = 0;
    qTarget = 0;
    active = false;
end
c=direction*c;
% 이동이 끝난 상태에서 새 접촉 방향이 들어오면 목표각 갱신
if ~active && c ~= 0 && c ~= cPrev
    qStart = qTarget;

    if c == 1
        qTarget = dTheta;
    elseif c == -1
        qTarget = 0;
    end

    elapsed = 0;
    active = true;
end

cPrev = c;

if active
    r = min(elapsed/Tp, 1);
    qcmd = qStart + r*(qTarget - qStart);
    elapsed = elapsed + Ts;

    if r >= 1
        active = false;
    end
else
    qcmd = qTarget;
end

== matlab function Quadruped_view/Quadruped Robot/Sensors/UpperBody Sensors/MATLAB Function2 ==
  data: q input; direction output
function direction= getHeading(q)
qw = q(1);
qx = q(2);
qy = q(3);
qz = q(4);

h = 2*(qw*qy - qx*qz);
direction = sign(h);
end
